simulink library "actuatorsLibrary"  (R2026a)
settings: Solver=ode45  EnableMultiTasking=on
libraries: aerolibactuator x2
settings Model: Creator=The MathWorks, Inc.  LastModifiedBy=The MathWorks, Inc.
settings DebuggingCC: SymbolicDimsDataTypeCodeGenerationDiagnostic=none
settings HardwareCC: ProdHWDeviceType=32-bit Generic

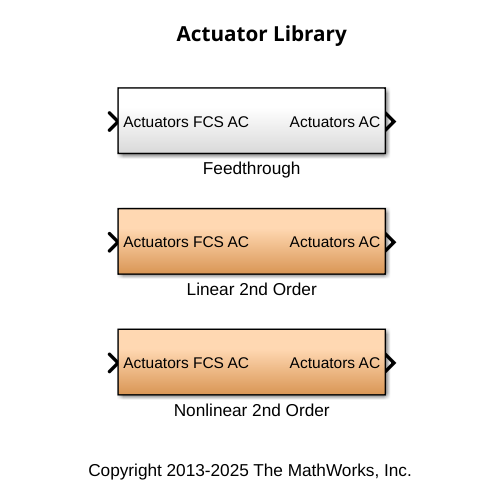
[thumbnail: Simulink's stored preview of the top-level diagram]
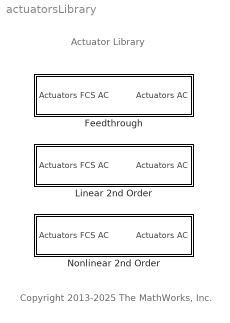
== system actuatorsLibrary ==
  note: Actuator Library
  note: Copyright 2013-2025 The MathWorks, Inc.
  Feedthrough : Subsystem  VariantControl=Variants.Actuators == 0
  Linear 2nd Order : Subsystem  VariantControl=Variants.Actuators == 1
  Nonlinear 2nd Order : Subsystem  VariantControl=Variants.Actuators == 2

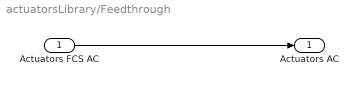
== system actuatorsLibrary/Feedthrough ==
  Actuators FCS AC : Inport
  Actuators AC : Outport  VectorParamsAs1DForOutWhenUnconnected=off
  wires:
  Actuators FCS AC/1 -> Actuators AC/1

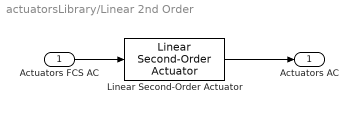
== system actuatorsLibrary/Linear 2nd Order ==
  Actuators FCS AC : Inport
  Linear Second-Order Actuator : aerolibactuator/Linear Second-Order Actuator  wn_fin=Vehicle.Nonlinear.Nonlinear.ACModel.Actuator.Linear.natFreq  z_fin=Vehicle.Nonlinear.Nonlinear.ACModel.Actuator.Linear.damping  fin_act_0=Vehicle.Nonlinear.Nonlinear.ACModel.Actuator.Linear.initPosition  fin_act_vel=Vehicle.Nonlinear.Nonlinear.ACModel.Actuator.Linear.initVelocity
  Actuators AC : Outport  VectorParamsAs1DForOutWhenUnconnected=off
  wires:
  Actuators FCS AC/1 -> Linear Second-Order Actuator/1
  Linear Second-Order Actuator/1 -> Actuators AC/1

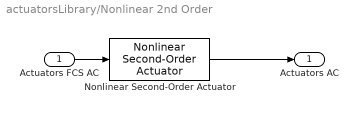
== system actuatorsLibrary/Nonlinear 2nd Order ==
  Actuators FCS AC : Inport
  Nonlinear Second-Order Actuator : aerolibactuator/Nonlinear Second-Order Actuator  wn_fin=Vehicle.Nonlinear.Nonlinear.ACModel.Actuator.NonLinear.natFreq  z_fin=Vehicle.Nonlinear.Nonlinear.ACModel.Actuator.NonLinear.damping  fin_max=Vehicle.Nonlinear.Nonlinear.ACModel.Actuator.NonLinear.maxDeflection  fin_min=Vehicle.Nonlinear.Nonlinear.ACModel.Actuator.NonLinear.minDeflection  fin_maxrate=Vehicle.Nonlinear.Nonlinear.ACModel.Actuator.NonLinear.rateLimit  fin_act_0=Vehicle.Nonlinear.Nonlinear.ACModel.Actuator.NonLinear.initPosition  fin_act_vel=Vehicle.Nonlinear.Nonlinear.ACModel.Actuator.NonLinear.initVelocity
  Actuators AC : Outport  VectorParamsAs1DForOutWhenUnconnected=off
  wires:
  Actuators FCS AC/1 -> Nonlinear Second-Order Actuator/1
  Nonlinear Second-Order Actuator/1 -> Actuators AC/1
